simulink model "fuzzy_cntrler"  (R2025b)
settings: Solver=FixedStepDiscrete  StartTime=0.0  StopTime=15  FixedStep=5e-6  MaxStep=5e-6  RelTol=1e-3
model workspace (MAT data in the model file):
  fxpopt_stateflow_dt_s206_g4 : handle (value not decoded)
  fxpopt_stateflow_dt_s207_g5 : handle (value not decoded)
undefined symbols (not defined in the file): Ion, Lithium
libraries: spsSeriesRLCBranchLib x12, spsMosfetLib x12, spsCurrentMeasurementLib x3, spsBatteryLib x2, spsLinearTransformerLib x1, dspstat3 x1, simulink x1, hdlsllib x1, fuzblock x1, spsVoltageMeasurementLib x1, sps_lib x1
settings Model: DataTypeOverride=Off  MinMaxOverflowLogging=ForceOff  MinMaxOverflowArchiveMode=Merge  FPTRunName=fxpOptimization.BaselineRun  SimulationMode=accelerator  Creator=tanuj  LastModifiedBy=tanuj
settings SolverCC: ZeroCrossControl=DisableAll  ZeroCrossAlgorithm=Adaptive  AutoInsertRateTranBlk=on
settings DataIOCC: SaveOutput=off  SaveTime=off  Refine=2
settings OptimizationCC: BlockReduction=off  ConditionallyExecuteInputs=off
settings DebuggingCC: MaskedZcDiagnostic=none  IgnoredZcDiagnostic=none  MultiTaskCondExecSysMsg=warning  SingleTaskRateTransMsg=warning  IntegerOverflowMsg=none  ParameterDowncastMsg=none  ParameterOverflowMsg=none  ParameterPrecisionLossMsg=none  IntegerSaturationMsg=none

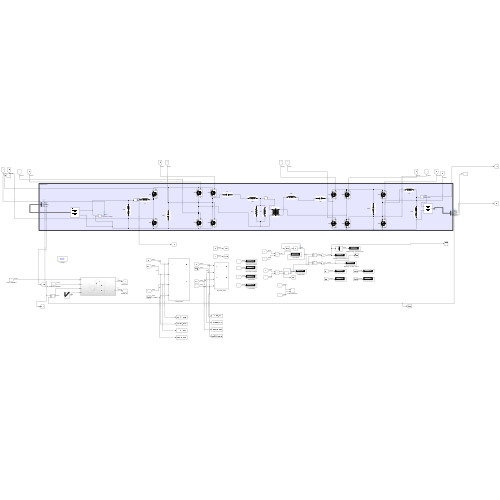
[thumbnail: Simulink's stored preview of the top-level diagram]
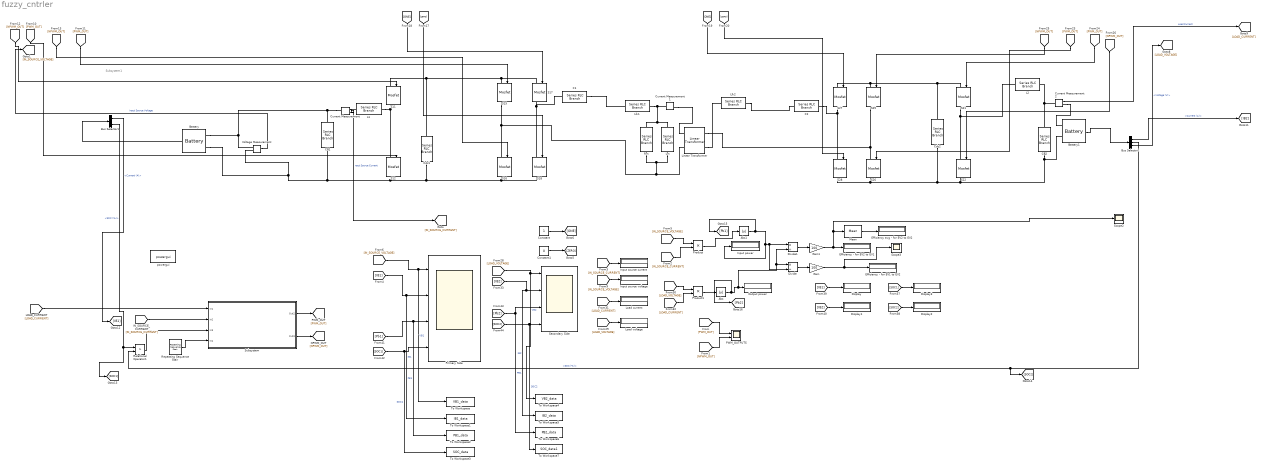
== system fuzzy_cntrler ==
  note: Subsystem1
  Abs : Abs  SaturateOnIntegerOverflow=off
  Abs1 : Abs  SaturateOnIntegerOverflow=off
  Battery : spsBatteryLib/Battery  BatType=Lithium-Ion  NomV=350  NomQ=60  SOC=75  Batt_Tr=30  PresetModel=on  MaxQ=60  MinV=262.5  FullV=407.3955  Dis_rate=26.087  R=0.058333  Normal_OP=54.2609  expZone="[378.135      2.947826]"
  Battery1 : spsBatteryLib/Battery  BatType=Lithium-Ion  NomV=450  NomQ=80  SOC=25  Batt_Tr=30  PresetModel=off  MaxQ=80  MinV=337.5  FullV=523.7942  Dis_rate=34.7826  R=0.05625  Normal_OP=72.3478  expZone="[486.1736      3.930435]"
  Bus Selector1 : BusSelector  OutputSignals=Current (A),SOC (%)
  Bus Selector2 : BusSelector  OutputSignals=Current (A),SOC (%),Voltage (V)
  "C1 " : spsSeriesRLCBranchLib/Series RLC Branch  LConnTagsString=__new0  RConnTagsString=__new0  BranchType=C  Resistance=1  Inductance=1e-3  SetiL0=off  InitialCurrent=0  Capacitance=0.21e-3  Setx0=off  InitialVoltage=0  Measurements=None
  C2 : spsSeriesRLCBranchLib/Series RLC Branch  LConnTagsString=__new0  RConnTagsString=__new0  BranchType=C  Resistance=1  Inductance=1e-3  SetiL0=off  InitialCurrent=0  Capacitance=0.21e-3  Setx0=off  InitialVoltage=0  Measurements=None
  CB1 : spsSeriesRLCBranchLib/Series RLC Branch  LConnTagsString=__new0  RConnTagsString=__new0  BranchType=RC  Resistance=0.01  Inductance=1e-3  SetiL0=off  InitialCurrent=0  Capacitance=1.6e-6  Setx0=off  InitialVoltage=350  Measurements=None
  CB2 : spsSeriesRLCBranchLib/Series RLC Branch  LConnTagsString=__new0  RConnTagsString=__new0  BranchType=RC  Resistance=0.01  Inductance=1e-3  SetiL0=off  InitialCurrent=0  Capacitance=1.8e-6  Setx0=off  InitialVoltage=0  Measurements=None
  Cdc1 : spsSeriesRLCBranchLib/Series RLC Branch  LConnTagsString=__new0  RConnTagsString=__new0  BranchType=C  Resistance=1  Inductance=1e-3  SetiL0=off  InitialCurrent=0  Capacitance=0.5e-3  Setx0=off  InitialVoltage=350  Measurements=None
  Cdc2 : spsSeriesRLCBranchLib/Series RLC Branch  LConnTagsString=__new0  RConnTagsString=__new0  BranchType=C  Resistance=1  Inductance=1e-3  SetiL0=off  InitialCurrent=0  Capacitance=0.8e-3  Setx0=off  InitialVoltage=450  Measurements=None
  Constant : Constant
  Constant1 : Constant  Value=0
  Current Measurement : spsCurrentMeasurementLib/Current Measurement  PhasorSimulation=off  OutputType=Complex  PSBequivalent=0
  Current Measurement1 : spsCurrentMeasurementLib/Current Measurement  PhasorSimulation=off  OutputType=Complex  PSBequivalent=0
  Current Measurement2 : spsCurrentMeasurementLib/Current Measurement  PhasorSimulation=off  OutputType=Complex  PSBequivalent=0
  Display{,1..3} (4 alike) : Display
  Divide : Product  Inputs=*/
  Divide1 : Product  Inputs=*/
  Efficiency - for EV1 to EV2 : Display
  Efficiency - for EV2 to EV1 : Display
  Efficiency avg - for EV2 to EV2 : Display
  Gain : Gain  Gain=100
  Gain1 : Gain  Gain=100
  Input power : Display
  Input source current : Display
  Input source voltage : Display
  L1 : spsSeriesRLCBranchLib/Series RLC Branch  LConnTagsString=__new0  RConnTagsString=__new0  BranchType=L  Resistance=1  Inductance=1.11e-3  SetiL0=off  InitialCurrent=0  Capacitance=1e-6  Setx0=off  InitialVoltage=0  Measurements=None
  L2 : spsSeriesRLCBranchLib/Series RLC Branch  LConnTagsString=__new0  RConnTagsString=__new0  BranchType=L  Resistance=1  Inductance=1.15e-3  SetiL0=off  InitialCurrent=40  Capacitance=1e-6  Setx0=off  InitialVoltage=0  Measurements=None
  Linear Transformer : spsLinearTransformerLib/Linear Transformer  UNITS=pu  NominalPower=[24000 50000]  winding1=[350 0.02 0.01]  winding2=[450 0.002 0.01]  ThreeWindings=off  winding3=[ 315e3 0.002 0.08 ]  RmLm=[500 500]  Measurements=None  DataType=off
  Llk1 : spsSeriesRLCBranchLib/Series RLC Branch  LConnTagsString=__new0  RConnTagsString=__new0  BranchType=L  Resistance=1  Inductance=0.3015e-6  SetiL0=off  InitialCurrent=0  Capacitance=1e-6  Setx0=off  InitialVoltage=0  Measurements=None
  Llk2 : spsSeriesRLCBranchLib/Series RLC Branch  LConnTagsString=__new0  RConnTagsString=__new0  BranchType=L  Resistance=1  Inductance=0.3015e-6  SetiL0=off  InitialCurrent=0  Capacitance=1e-6  Setx0=off  InitialVoltage=0  Measurements=None
  Lm : spsSeriesRLCBranchLib/Series RLC Branch  LConnTagsString=__new0  RConnTagsString=__new0  BranchType=L  Resistance=1  Inductance=2.2725e-3  SetiL0=off  InitialCurrent=0  Capacitance=1e-6  Setx0=off  InitialVoltage=0  Measurements=None
  Load current : Display
  Load voltage : Display
  Mean : dspstat3/Mean  run=off  InputProcessing=Columns as channels (frame based)  reset_popup=None  directionMode=Each column  dimension=1  roiEnable=off  roiType=Rectangles  roiPortion=Entire ROI  roiOutput=Individual statistics for each ROI  roiFlag=off  roundingMode=Floor  overflowMode=off  outputDataTypeStr=Inherit: Same as accumulator  outputMin=[]  outputMax=[]  outputLastDataTypeStr=Inherit: Same as accumulator
  Output power : Display
  PWM_OUTPUTS : Scope  NumInputPorts=2
      settings: ActiveDisplayYMinimum=-0.125  ActiveDisplayYMaximum=1.125  DataLoggingVariableName=ScopeData3
  Primary Side : Scope  NumInputPorts=4
      settings: ActiveDisplayString=4  ActiveDisplayYMinimum=75.749575486279724  ActiveDisplayYMaximum=75.8301030461193
  Product : Product
  Product1 : Product
  Relational Operator1 : RelationalOperator  Operator=>  OutDataTypeStr=boolean  RndMeth=Simplest  InputSameDT=off
  Repeating Sequence Stair : simulink/Sources/Repeating Sequence Stair  OutValues=[10 20 30 40 50].'  tsamp=3  OutMin=[]  OutMax=[]  OutDataTypeStr=double  OutputDataTypeScalingMode=double  OutDataType=fixdt(1,16,3)  ConRadixGroup=Best Precision: Vector-wise  OutScaling=[]
  Rm : spsSeriesRLCBranchLib/Series RLC Branch  LConnTagsString=__new0  RConnTagsString=__new0  BranchType=R  Resistance=500  Inductance=1e-3  SetiL0=off  InitialCurrent=0  Capacitance=1e-6  Setx0=off  InitialVoltage=0  Measurements=None
  S{11..12,15..17,21..22,25..28} (11 alike) : spsMosfetLib/Mosfet  Ron=0.1  Lon=0  Rd=0.01  Vfd=0  IC=0  Rs=1e5  Cs=inf  Measurements=on
  S18 : spsMosfetLib/Mosfet  Ron=0.2  Lon=0  Rd=0.2  Vfd=0  IC=0  Rs=1e5  Cs=inf  Measurements=on
  Scope2 : Scope
  Scope3 : Scope
  Secondary Side : Scope  NumInputPorts=4
      settings: ActiveDisplayString=4  ActiveDisplayYMinimum=75.787524765681354  ActiveDisplayYMaximum=75.825886459519126
  Subsystem : Subsystem
  To Workspace : ToWorkspace  VariableName=VB1_data  SaveFormat=Timeseries  SampleTime=-1
  To Workspace1 : ToWorkspace  VariableName=IB1_data  SaveFormat=Timeseries  SampleTime=-1
  To Workspace2 : ToWorkspace  VariableName=PB1_data  SaveFormat=Timeseries  SampleTime=-1
  To Workspace3 : ToWorkspace  VariableName=SOC_data  SaveFormat=Timeseries  SampleTime=-1
  To Workspace4 : ToWorkspace  VariableName=VB2_data  SaveFormat=Timeseries  SampleTime=-1
  To Workspace5 : ToWorkspace  VariableName=IB2_data  SaveFormat=Timeseries  SampleTime=-1
  To Workspace6 : ToWorkspace  VariableName=PB2_data  SaveFormat=Timeseries  SampleTime=-1
  To Workspace7 : ToWorkspace  VariableName=SOC_data1  SaveFormat=Timeseries  SampleTime=-1
  Voltage Measurement : spsVoltageMeasurementLib/Voltage Measurement  PhasorSimulation=off  OutputType=Complex  PSBequivalent=0
  powergui : sps_lib/powergui  Priority=1  SimulationMode=Discrete  SampleTime=5e-6  frequency=60  Iterations=50  frequencyindice=0  Pbase=100e6  ErrMax=1e-4  UnitsV=kV  UnitsW=MW  buscounter=0  FunctionMessages=off  echomessages=off  EnableUseOfTLC=off  CurrentSourceSwitches=off  DisableSnubberDevices=off  DisableRonSwitches=off  DisableVfSwitches=off  DisplayEquations=off  AutomaticDiscreteSolvers=off  SolverType=Tustin/Backward Euler (TBE)  Interpol=off  ExternalGateDelay=off  methode=off  Ts=100  x0status=blocks  SPID=on  SwTol=0  HookPort=off  NonlinearTolerance=1e-4  nMaxIteration=100  ContinueOnMaxIteration=off  RestoreLinks=warning  ResistiveCurrentMeasurement=off  Frange=[0:2:500]  Ylog=off  Xlog=on  ShowGrid=off  save=off  variable=ZData  structure=0  ZoomFFT=off  StartTime=0.0  cycles=1  DisplayStyle=1  fundamental=60  FreqAxis=off  MaxFrequency=1000  frequencyindicesteady=1  RmsSteady=1  display=off
  wires:
  Product/1 -> Abs1/1
  Product1/1 -> Abs/1
  [PWM_OUT] -> PWM_OUTPUTS/1
  [NPWM_OUT] -> PWM_OUTPUTS/2
  [IN_SOURCE_CURRENT] -> Product/2
  [IN_SOURCE_CURRENT] -> Input source current/1
  [IB1] -> To Workspace1/1, Primary Side/2  "IB1"
  [IN_SOURCE_VOLTAGE] -> Product/1
  [IN_SOURCE_VOLTAGE] -> To Workspace/1, Primary Side/1  "VB1"
  [IN_SOURCE_VOLTAGE] -> Input source voltage/1
  Constant1/1 -> [ZERO]
  Constant/1 -> [ONE]
  [LOAD_VOLTAGE] -> Load voltage/1
  [LOAD_VOLTAGE] -> Product1/1
  [LOAD_CURRENT] -> Load current/1
  [LOAD_CURRENT] -> Product1/2
  [IB2] -> Secondary Side/2, To Workspace5/1  "IB2"
  [LOAD_VOLTAGE] -> To Workspace4/1, Secondary Side/1  "VB2"
  Divide/1 -> Gain/1
  [SOC1] -> Display3/1
  [SOC2] -> Display2/1
  [IB1] -> Display/1
  [IB2] -> Display1/1
  [Pb1] -> To Workspace2/1, Primary Side/3  "PB1"
  [SOC1] -> To Workspace3/1, Primary Side/4  "SOC1"
  [Pb2] -> Secondary Side/3, To Workspace6/1  "PB1"
  [SOC2] -> To Workspace7/1, Secondary Side/4  "SOC2"
  Divide1/1 -> Gain1/1
  Gain1/1 -> Mean/1, Scope2/1, Efficiency - for EV2 to EV1/1
  Abs/1 -> [Pb2], Divide/1, Divide1/2, Output power/1
  Abs1/1 -> Divide/2, Divide1/1, Input power/1, [Pb1]
  Gain/1 -> Scope3/1, Efficiency - for EV1 to EV2/1
  Mean/1 -> Efficiency avg - for EV2 to EV2/1
  Relational Operator1/1 -> Subsystem/3(In3)
  Subsystem/1(Out2) -> [PWM_OUT]
  Subsystem/2(Out3) -> [NPWM_OUT]
  Voltage Measurement/1 -> [IN_SOURCE_VOLTAGE]  "Input Source Voltage"
  [NPWM_OUT] -> S25/1
  [PWM_OUT] -> S15/1
  [PWM_OUT] -> S21/1
  [NPWM_OUT] -> S11/1
  Bus Selector2/2 -> Relational Operator1/2, [SOC2]  "<SOC (%)>"
  Bus Selector2/1 -> [IB2]  "<Current (A)>"
  Bus Selector1/2 -> [SOC1], Relational Operator1/1  "<SOC (%)>"
  [ZERO] -> S18/1
  [PWM_OUT] -> S26/1
  [PWM_OUT] -> S12/1
  [NPWM_OUT] -> S16/1
  Bus Selector1/1 -> [IB1]  "<Current (A)>"
  Bus Selector2/3 -> [LOAD_VOLTAGE]  "<Voltage (V)>"
  [NPWM_OUT] -> S22/1
  [ONE] -> S27/1
  Current Measurement/1 -> [IN_SOURCE_CURRENT]  "nput Source Current"
  Battery/1 -> Bus Selector1/1
  [ONE] -> S17/1
  [ZERO] -> S28/1
  Current Measurement2/1 -> [LOAD_CURRENT]  "Load Current"
  Battery1/1 -> Bus Selector2/1
  [LOAD_CURRENT] -> Subsystem/1(In1)
  [IN_SOURCE_CURRENT] -> Subsystem/2(In2)
  Repeating Sequence Stair/1 -> Subsystem/4(In4)
  connections:
  S17/RConn1 -- "C1 "/RConn1 -- S18/LConn1
  "C1 "/LConn1 -- Llk1/LConn1
  S25/RConn1 -- Linear Transformer/RConn1 -- S26/LConn1
  Llk2/LConn1 -- C2/LConn1
  Linear Transformer/RConn2 -- Llk2/RConn1
  S27/RConn1 -- C2/RConn1 -- S28/LConn1
  Current Measurement/RConn1 -- L1/LConn1
  S27/LConn1 -- S25/LConn1 -- Cdc2/LConn1 -- S21/LConn1
  Current Measurement1/RConn1 -- Linear Transformer/LConn1
  S11/RConn1 -- L1/RConn1 -- S12/LConn1
  S15/RConn1 -- Linear Transformer/LConn2 -- Lm/RConn1 -- Rm/RConn1 -- S16/LConn1
  Current Measurement/LConn1 -- Voltage Measurement/LConn1 -- Battery/LConn1 -- CB1/LConn1
  S17/LConn1 -- S15/LConn1 -- S11/LConn1 -- Cdc1/LConn1
  S12/RConn1 -- Cdc1/RConn1 -- S18/RConn1 -- S16/RConn1 -- Battery/LConn2 -- Voltage Measurement/LConn2 -- CB1/RConn1
  Rm/LConn1 -- Llk1/RConn1 -- Current Measurement1/LConn1 -- Lm/LConn1
  CB2/LConn1 -- Current Measurement2/LConn1 -- L2/RConn1
  S21/RConn1 -- L2/LConn1 -- S22/LConn1
  S28/RConn1 -- S26/RConn1 -- Cdc2/RConn1 -- Battery1/LConn2 -- CB2/RConn1 -- S22/RConn1
  Current Measurement2/RConn1 -- Battery1/LConn1

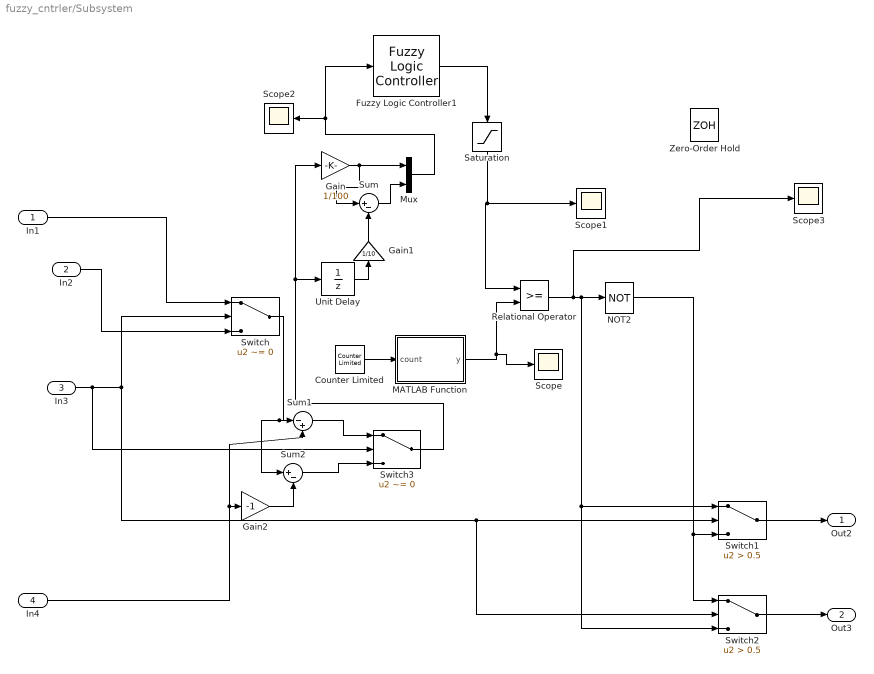
== system fuzzy_cntrler/Subsystem ==
  In1 : Inport  SampleTime=5e-6
  In2 : Inport  Port=2  SampleTime=5e-6
  In3 : Inport  Port=3  SampleTime=5e-6
  In4 : Inport  Port=4  SampleTime=5e-6
  Counter Limited : hdlsllib/Sources/Counter Limited  uplimit=7  tsamp=5e-6
  Fuzzy Logic Controller1 : fuzblock/Fuzzy Logic  Controller  FIS=ev_v2v  OutputSampleNumber=101  DataType=double  UseLookupTable=on  NumBreakpoints=10  FuzzifiedInputs=off  RuleFiringStrengths=off  RuleOutputs=off  AggregatedOutputs=off  SimulateUsing=Interpreted execution  OutOfRangeInputValueMessage=warning  NoRuleFiredMessage=warning  EmptyOutputFuzzySetMessage=warning
  Gain : Gain  Gain=1/100
  Gain1 : Gain  Gain=1/10
  Gain2 : Gain  Gain=-1  ParamDataTypeStr=double  OutDataTypeStr=double
  MATLAB Function : MATLAB Function  TreatAsAtomicUnit=on
  Mux : Mux  Inputs=2
  NOT2 : Logic  Operator=NOT  IconShape=distinctive  AllPortsSameDT=off  OutDataTypeStr=boolean
  Relational Operator : RelationalOperator  OutDataTypeStr=boolean  RndMeth=Simplest  InputSameDT=off
  Saturation : Saturate  LowerLimit=0.3
  Scope{,1..3} (4 alike) : Scope
      Scope settings: ActiveDisplayYMinimum=-0.125  ActiveDisplayYMaximum=1.125  DataLoggingVariableName=ScopeData2
      Scope1 settings: ActiveDisplayYMinimum=0.37596130682062812  ActiveDisplayYMaximum=0.61634823861434651
      Scope2 settings: ActiveDisplayYMinimum=-68.665527036967717  ActiveDisplayYMaximum=519.05187231457091  DataLoggingVariableName=ScopeData4
      Scope3 settings: ActiveDisplayYMinimum=-0.032969344673656753  ActiveDisplayYMaximum=1.018021399957612  DataLoggingVariableName=ScopeData5
  Sum : Sum  Inputs=|+-
  Sum1 : Sum  Inputs=|-+  OutDataTypeStr=double  AccumDataTypeStr=double
  Sum2 : Sum  Inputs=|+-  OutDataTypeStr=double  AccumDataTypeStr=double
  Switch : Switch  Criteria=u2 ~= 0  Threshold=0.5  OutDataTypeStr=double  SaturateOnIntegerOverflow=off  InputSameDT=off
  Switch1 : Switch  Criteria=u2 > Threshold  Threshold=0.5  SaturateOnIntegerOverflow=off  InputSameDT=off
  Switch2 : Switch  Criteria=u2 > Threshold  Threshold=0.5  SaturateOnIntegerOverflow=off  InputSameDT=off
  Switch3 : Switch  Criteria=u2 ~= 0  Threshold=0.5  OutDataTypeStr=double  SaturateOnIntegerOverflow=off  InputSameDT=off
  Unit Delay : UnitDelay  SampleTime=-1  HasFrameUpgradeWarning=on
  Zero-Order Hold : ZeroOrderHold  SampleTime=1e-4
  Out2 : Outport  SampleTime=5e-6
  Out3 : Outport  Port=2  SampleTime=5e-6
  wires:
  In3/1 -> Switch2/2, Switch1/2, Switch/2, Switch3/2
  Relational Operator/1 -> Scope3/1, Switch2/3, Switch1/1, NOT2/1
  Switch/1 -> Sum2/1, Sum1/1
  In4/1 -> Sum1/2, Gain2/1
  Gain2/1 -> Sum2/2
  Switch2/1 -> Out3/1
  Sum1/1 -> Switch3/1
  NOT2/1 -> Switch2/1, Switch1/3
  In1/1 -> Switch/1
  Sum2/1 -> Switch3/3
  In2/1 -> Switch/3
  Switch1/1 -> Out2/1
  MATLAB Function/1(y) -> Scope/1, Relational Operator/2
  Sum/1 -> Mux/2
  Mux/1 -> Fuzzy Logic Controller1/1, Scope2/1
  Switch3/1 -> Gain/1, Unit Delay/1
  Unit Delay/1 -> Gain1/1
  Gain/1 -> Sum/1, Mux/1
  Gain1/1 -> Sum/2
  Fuzzy Logic Controller1/1 -> Saturation/1
  Counter Limited/1 -> MATLAB Function/1(count)
  Saturation/1 -> Relational Operator/1, Scope1/1

== matlab function fuzzy_cntrler/Subsystem/MATLAB Function ==
  data: count input; y output
function y = fcn(count)
%#codegen
% Triangle wave - original working version
% count: uint8 from Counter Limited (0 to 7)
% y: double [0,1]

N      = uint8(8);
HALF_N = uint8(4);
c      = uint8(count);

if c < HALF_N
    y = double(c) / double(HALF_N);
else
    y = double(N - c) / double(HALF_N);
end
